simulink model "sf_loop_scheduler"  (R2025b)
settings: Solver=FixedStepDiscrete  StartTime=0.0  StopTime=10  RelTol=1e-3  EnableMultiTasking=on
model workspace (MAT data in the model file):
  deltat = 0.001
settings Model: Creator=The MathWorks, Inc.  LastModifiedBy=The MathWorks, Inc.
settings SolverCC: AlgebraicLoopSolver=TrustRegion  InsertRTBMode=Auto
settings DataIOCC: SaveFormat=Array  ReturnWorkspaceOutputs=off
settings OptimizationCC: ReuseModelBlockBuffer=off  ExpressionDepthLimit=2147483647.0  InitFltsAndDblsToZero=on  LifeSpan=inf
settings DebuggingCC: SaveWithParameterizedLinksMsg=none  UnderspecifiedInitializationDetection=Classic  MergeDetectMultiDrivingBlocksExec=none  SignalResolutionControl=TryResolveAllWithWarning  InheritedTsInSrcMsg=none  MultiTaskDSMMsg=warning  MultiTaskCondExecSysMsg=none  FcnCallInpInsideContextMsg=warning  UnconnectedInputMsg=warning  UnconnectedOutputMsg=warning  UnconnectedLineMsg=warning  StateNameClashWarn=warning  SFUnexpectedBacktrackingDiag=warning  SFNoUnconditionalDefaultTransitionDiag=warning  SFExecutionAtInitializationDiag=none  ArithmeticOperatorsInVariantConditions=warning
settings HardwareCC: ProdBitPerPointer=32.0  ProdBitPerSizeT=32.0  ProdBitPerPtrDiffT=32.0  ProdLargestAtomicFloat=None  ProdIntDivRoundTo=Undefined  ProdEndianess=Unspecified  ProdWordSize=32.0  ProdHWDeviceType=32-bit Generic
settings ModelReferenceCC: EnableRefExpFcnMdlSchedulingChecks=on  PropagateSignalLabelsOutOfModel=off
settings SFSimCC: SFSimEcho=off  SimUseLocalCustomCode=off  SimParseCustomCode=off
settings RTWCC: RTWUseLocalCustomCode=off  GPUComputeCapability=3.5
settings CodeAppCC: StateflowObjectComments=on
settings GRTTargetCC: TargetFcnLib=ansi_tfl_tmw.mat  TargetLangStandard=C89/C90 (ANSI)  CombineOutputUpdateFcns=off  GRTInterface=on
settings ConfigComp: CovMetricSettings=dw  CovSaveCumulativeToWorkspaceVar=on  CovSaveSingleToWorkspaceVar=on  CovExternalEMLEnable=off  CovSFcnEnable=off

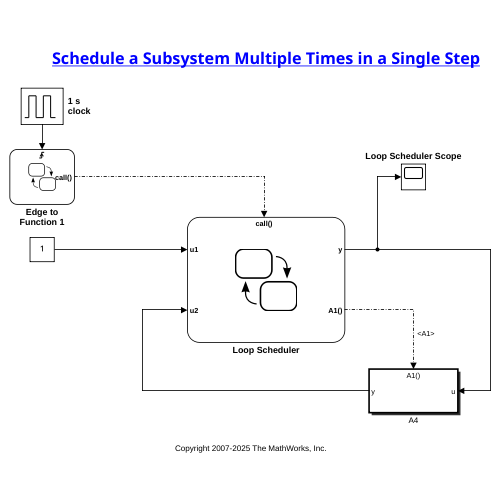
[thumbnail: Simulink's stored preview of the top-level diagram]
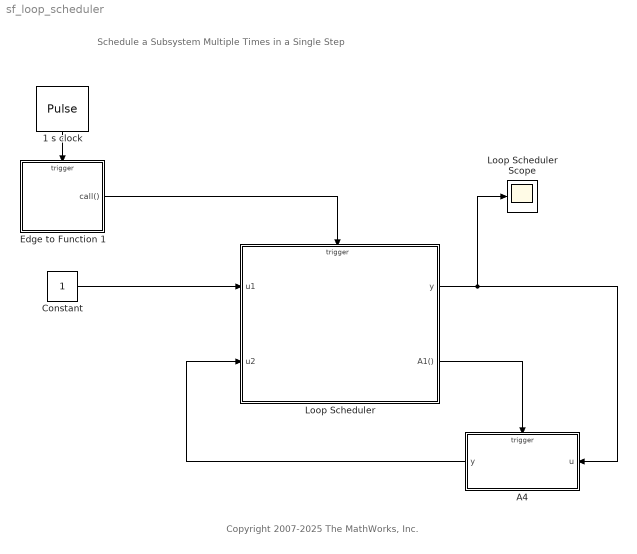
== system sf_loop_scheduler ==
  note: Copyright 2007-2025 The MathWorks, Inc.
  note: Schedule a Subsystem Multiple Times in a Single Step
  1 s clock : DiscretePulseGenerator  PulseType=Time based  Period=1  PulseWidth=10
  A4 : Subsystem  TreatAsAtomicUnit=on
  Constant : Constant
  Edge to Function 1 : Stateflow chart  TreatAsAtomicUnit=on
  Loop Scheduler : Stateflow chart  TreatAsAtomicUnit=on
  Loop Scheduler Scope : Scope
      settings: TimeSpan=10  ActiveDisplayYMinimum=-31.0625  ActiveDisplayYMaximum=279.5625
  wires:
  Loop Scheduler/1(y) -> A4/1(u), Loop Scheduler Scope/1
  1 s clock/1 -> Edge to Function 1/Trigger
  Edge to Function 1/1(call()) -> Loop Scheduler/Trigger
  Loop Scheduler/2(A1()) -> A4/Trigger
  A4/1(y) -> Loop Scheduler/2(u2)
  Constant/1 -> Loop Scheduler/1(u1)

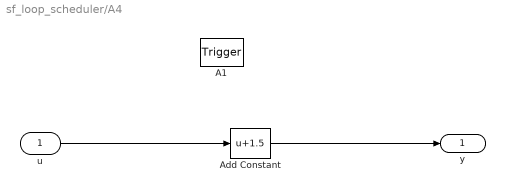
== system sf_loop_scheduler/A4 ==
  u : Inport
  A1 : TriggerPort  TriggerType=function-call  VariantControl=Variant
  Add Constant : Bias  Bias=1.5  SaturateOnIntegerOverflow=off
  y : Outport  VectorParamsAs1DForOutWhenUnconnected=off
  wires:
  u/1 -> Add Constant/1
  Add Constant/1 -> y/1

== stateflow chart sf_loop_scheduler/Edge to Function 1 ==
  settings: executeAtInitialization=1
  (default) -> (junction 2) : {call;}
  events: edge input RISING_EDGE_EVENT; call output FUNCTION_CALL_EVENT

== stateflow chart sf_loop_scheduler/Loop Scheduler ==
  settings: executeAtInitialization=1
  (default) -> (junction 5) : {i=1;}
  (junction 6) -> (junction 5) [order 1] : [i<=10]
      | {
      | send(A1);
      | y = u1+u2;
      | i++;
      | }
  (junction 5) -> (junction 6)
  (junction 6) -> (junction 7) [order 2] : // done
  data: y output double; u1 input; u2 input; i local uint32
  events: A1 output FUNCTION_CALL_EVENT; call input FUNCTION_CALL_EVENT
